simulink model "Three_Phase_Full_Wave"  (R2025b)
settings: Solver=VariableStepAuto  StartTime=0.0  StopTime=10.0  RelTol=1e-3
libraries: fl_lib x10, nesl_utility x9, ee_lib x8
settings Model: Creator=USER  LastModifiedBy=USER

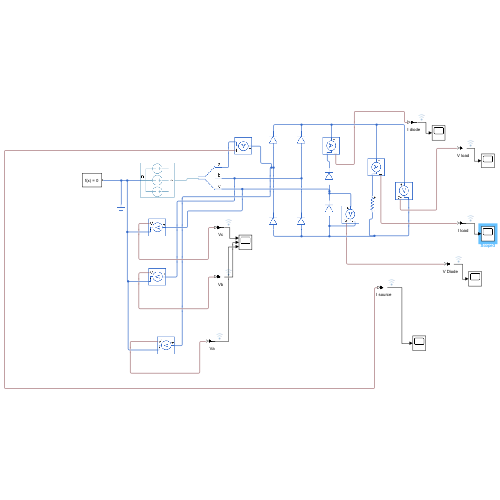
[thumbnail: Simulink's stored preview of the top-level diagram]
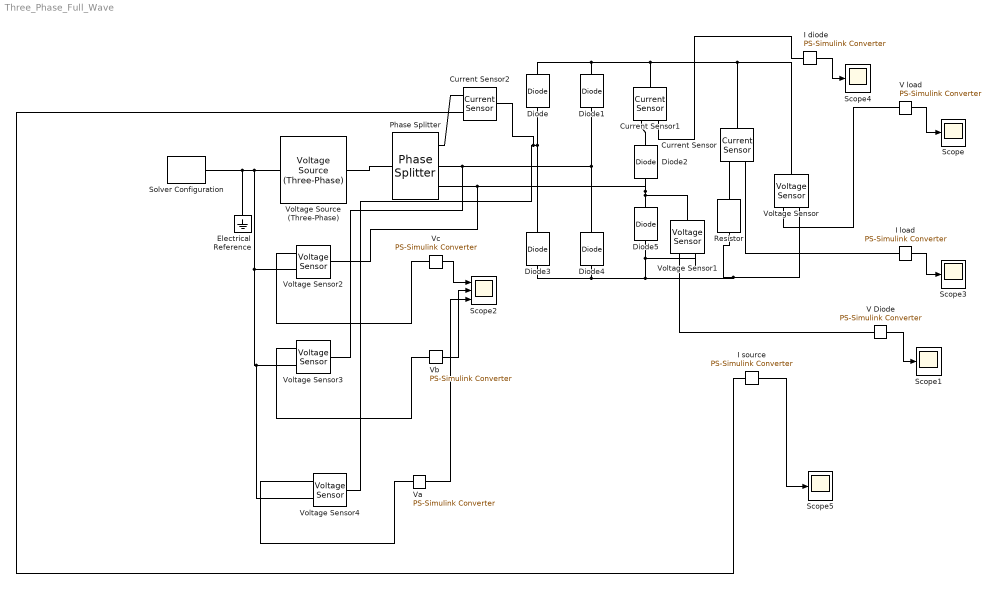
== system Three_Phase_Full_Wave ==
  Current Sensor : fl_lib/Electrical/Electrical Sensors/Current Sensor
  Current Sensor1 : fl_lib/Electrical/Electrical Sensors/Current Sensor
  Current Sensor2 : fl_lib/Electrical/Electrical Sensors/Current Sensor
  Diode{,1..5} (6 alike) : ee_lib/Semiconductors & Converters/Diode  ModelType=ee.enum.diode.modelType.pwl  TableType=ee.enum.diode.tableType.IfMat  IfMat=[.07, .12, .19, 1.75, 4.24, 7.32, 11.2; .16, .3, .72, 2.14, 5.02, 8.35, 13.12] A  VfMat=[.9, 1.15, 1.25, 1.5, 1.75, 2.17, 2.6, 2.85; .58, .68, .75, 1.1, 1.38, 1.77, 2.27, 2.7] V  TjVec=[25, 125] degC  VfVec=[.5, .7, .9, 1.3, 1.7, 2.1, 2.5] V  IfVec=[.1, .2, .5, 1, 2, 4, 7, 10] A  IrMat=[1e-06, 2e-06, 5e-06, 1e-05, 2.5e-05, 5e-05, .0001; 2e-06, 5e-06, 1e-05, 4e-05, 8e-05, .0002, .0005] A  VrMat=[10, 100, 200, 250, 300, 325, 350; 10, 70, 160, 220, 270, 300, 320] V  VrVec=[10, 20, 40, 50, 70, 80, 100] V  IrVec=[1e-06, 2e-06, 5e-06, 1e-05, 2e-05, 5e-05, .0001] A  Vf=0.6 V  Ron=0.3 Ohm  Goff=1e-8 S  prmExp=ee.enum.diode.expParam.useTwo  I12=[.0137, .545] A  V12=[.6, .7] V  RS=0 Ohm  Tmeas=298.15 K  IS=1e-12 A  ec=1  I1=0.0137 A  V1=0.6 V  N_series=1  N_parallel=1  ZenerEnable=false  Rz=0.3 Ohm  BV=inf V  C_param=ee.enum.diode.capParam.fixed  CJ=0 pF  CJ0=5 pF  Vvec=[.1, 10, 100] V  Cvec=[3.5, 1, .4] pF  VJ=1 V  Mgrad=0.5  FC=0.5  Q_param=ee.enum.diode.recoveryParam.off  iRM=-7.15 A  iF=4 A  didt=-750 A/us  trr_factor=3  trr=115 ns  Qrr=150 nA*s  Vr=-600 V  Ls=150 nH  Erec=0.03 J  TT=50 ns  tau=100 ns  T_param=ee.enum.diode.temperatureParam.off  Tdevice=298.15 K  I1_T2=0.245 A  V1_T2=0.5 V  IS_T2=1.25e-7 A  Tmeas2=125 degC  XTI_param=ee.enum.diode.xtiParam.pn  XTI=3  EG_param=ee.enum.diode.egapParam.material_si  EG=1.11 eV  dBVdT=0 V/K  enable_fault_input=simscape.enum.onoff.off  i_specify=off  i_priority=None  i=0 A  i_nominal_specify=off  i_nominal_value=1  i_nominal_unit=A  v_specify=off  v_priority=None  v=0 V  v_nominal_specify=off  v_nominal_value=1  v_nominal_unit=V  v_capacitor_specify=off  v_capacitor_priority=None  v_capacitor=0 V  v_capacitor_nominal_specify=off  v_capacitor_nominal_value=1  v_capacitor_nominal_unit=V  Qj_specify=off  Qj_priority=High  Qj=0 C  Qj_nominal_specify=off  Qj_nominal_value=1  Qj_nominal_unit=C  i_diode_specify=off  i_diode_priority=None  i_diode=0 A  i_diode_nominal_specify=off  i_diode_nominal_value=1  i_diode_nominal_unit=A  v_diode_specify=off  v_diode_priority=None  v_diode=0 V  v_diode_nominal_specify=off  v_diode_nominal_value=1  v_diode_nominal_unit=V  i_capacitor_specify=off  i_capacitor_priority=None  i_capacitor=0 A  i_capacitor_nominal_specify=off  i_capacitor_nominal_value=1  i_capacitor_nominal_unit=A  power_dissipated_specify=off  power_dissipated_priority=None  power_dissipated=0 W  power_dissipated_nominal_specify=off  power_dissipated_nominal_value=1  power_dissipated_nominal_unit=W  fidelity_level=ee.enum.diode.fidelity.includeChargeDyn  rec_loss_model=ee.enum.diode.reverseRecoveryModel.fixed  ErecVal=0 J  scaleWithIandV=true  ErecMat=zeros(2, 3) J  TjrecVec=[298.15, 398.15] K  IfrecVec=[.1, 1, 10] A  IrecVal=10 A  VrecVal=10 V  tFilter=1 / 1000 / 100 s  thermal_network_parameterization=ee.enum.thermalNetworkTopology.junctionCase  Rth=[0, 10] K/W  Rth_Cauer=[1, 3, 10] K/W  Rth_Foster=[.08, .14, .22, .16] K/W  thermal_mass_parameterization=ee.enum.thermalNetwork.timeconstant  thermal_mass=[0, 1] J/K  thermal_mass_Cauer=[.1, .3, 1] J/K  thermal_mass_Foster=[.001, .005, .05, .5] J/K  thermal_time_constant=[0, 10] s  thermal_time_constant_Cauer=[1, 3, 10] s  thermal_time_constant_Foster=[7e-05, .0007, .01, .08] s  thermal_mass_initial_temperatures=[25, 25] degC  thermal_mass_initial_temperatures_Cauer=[25, 25, 25] degC  junction_thermal_mass=0.01 J/K  Tvec_initial_Foster=[25, 25, 25, 25] degC  no_thermal_network=0  junction_temperature_specify=off  junction_temperature_priority=None  junction_temperature=25 degC  junction_temperature_nominal_specify=off  junction_temperature_nominal_value=1  junction_temperature_nominal_unit=degC
  Electrical Reference : fl_lib/Electrical/Electrical Elements/Electrical Reference
  I diode : nesl_utility/PS-Simulink Converter  PhysicalDomain=network_engine_domain  SubClassName=ps_output  LeftPortType=input  RightPortType=output  PseudoPeriodic=off  Frequencies=[]  VectorFormat=inherit  Unit=inherit  AffineConversion=off
  I load : nesl_utility/PS-Simulink Converter  PhysicalDomain=network_engine_domain  SubClassName=ps_output  LeftPortType=input  RightPortType=output  PseudoPeriodic=off  Frequencies=[]  VectorFormat=inherit  Unit=inherit  AffineConversion=off
  I source : nesl_utility/PS-Simulink Converter  PhysicalDomain=network_engine_domain  SubClassName=ps_output  LeftPortType=input  RightPortType=output  PseudoPeriodic=off  Frequencies=[]  VectorFormat=inherit  Unit=inherit  AffineConversion=off
  Phase Splitter : ee_lib/Connectors & References/Phase Splitter
  Resistor : fl_lib/Electrical/Electrical Elements/Resistor  R=200 Ohm  i_specify=off  i_priority=None  i=0 A  i_nominal_specify=off  i_nominal_value=1  i_nominal_unit=A  v_specify=off  v_priority=None  v=0 V  v_nominal_specify=off  v_nominal_value=1  v_nominal_unit=V
  Scope{,1,3..5} (5 alike) : Scope
      Scope settings: ActiveDisplayYMinimum=92.210744218018334  ActiveDisplayYMaximum=110.53269114341096
      Scope1 settings: ActiveDisplayYMinimum=-14.541376131026752  ActiveDisplayYMaximum=123.24187283383368
      Scope3 settings: ActiveDisplayYMinimum=0.45248228896029896  ActiveDisplayYMaximum=0.57237016067869884  DataLoggingVariableName=ScopeData3
      Scope4 settings: ActiveDisplayYMinimum=-14145.384322688979  ActiveDisplayYMaximum=22660.519081846294  DataLoggingVariableName=ScopeData4
      Scope5 settings: ActiveDisplayYMinimum=-14145.384322688979  ActiveDisplayYMaximum=22660.519081846294  DataLoggingVariableName=ScopeData5
  Scope2 : Scope  NumInputPorts=3
      settings: ActiveDisplayYMinimum=-79.551289054539069  ActiveDisplayYMaximum=79.551289048706238  DataLoggingVariableName=ScopeData2
  Solver Configuration : nesl_utility/Solver Configuration  PhysicalDomain=network_engine_domain  SubClassName=solver  LeftPortType=input  RightPortType=generic  Tones=[]  Harmonics=[]  SimulateNoise=off  Profile=off  UseLocalSampling=off  EnableSwitchedLinearOptims=on  FrequencyDomain=off  UseCCode=off  RelTol=0.001  AbsTol=0.001  MinStep=1e-09  ToWorkspace=off  RevertToSquareIcSolve=off  NumHomotopyIterations=100  PhasorMode=off  PhasorModeNumHarmonics=1  ConsistencySolver=NEWTON_XTOL_AFTER_FTOL  IndexReductionMethod=DerivativeReplacement  DoDC=off  ResidualTolerance=1e-09  ConsistencyTolSource=GLOBAL  ConsistencyAbsTol=0.001  ConsistencyRelTol=0.001  ConsistencyTolFactor=0.001  UseLocalSolver=off  LocalSolverChoice=NE_BACKWARD_EULER_ADVANCER  ResolveIndetEquations=on  FunctionEvalNumThread=1  LocalSolverSampleTime=0.001  DoFixedCost=off  MaxNonlinIter=3  MaxModeIter=2  ComputeImpulses=off  ImpulseIterations=2  LinearAlgebra=auto  LinearAlgebraNumThread=0  EquationFormulation=NE_TIME_EF  DelaysMemoryBudget=1024  AutomaticFiltering=on  FilteringTimeConstant=0.001  PartitionStorageMethod=AS_NEEDED  PartitionMemoryBudget=1024  PartitionMethod=ROBUST  MultibodyUseLocalSolver=off  MultibodyLocalSolverChoice=ODE1  MultibodyLocalSolverSampleTime=0.001
  V Diode : nesl_utility/PS-Simulink Converter  PhysicalDomain=network_engine_domain  SubClassName=ps_output  LeftPortType=input  RightPortType=output  PseudoPeriodic=off  Frequencies=[]  VectorFormat=inherit  Unit=inherit  AffineConversion=off
  V load : nesl_utility/PS-Simulink Converter  PhysicalDomain=network_engine_domain  SubClassName=ps_output  LeftPortType=input  RightPortType=output  PseudoPeriodic=off  Frequencies=[]  VectorFormat=inherit  Unit=inherit  AffineConversion=off
  Va : nesl_utility/PS-Simulink Converter  PhysicalDomain=network_engine_domain  SubClassName=ps_output  LeftPortType=input  RightPortType=output  PseudoPeriodic=off  Frequencies=[]  VectorFormat=inherit  Unit=inherit  AffineConversion=off
  Vb : nesl_utility/PS-Simulink Converter  PhysicalDomain=network_engine_domain  SubClassName=ps_output  LeftPortType=input  RightPortType=output  PseudoPeriodic=off  Frequencies=[]  VectorFormat=inherit  Unit=inherit  AffineConversion=off
  Vc : nesl_utility/PS-Simulink Converter  PhysicalDomain=network_engine_domain  SubClassName=ps_output  LeftPortType=input  RightPortType=output  PseudoPeriodic=off  Frequencies=[]  VectorFormat=inherit  Unit=inherit  AffineConversion=off
  Voltage Source (Three-Phase) : ee_lib/Sources/Voltage Source (Three-Phase)  vline_rms=sqrt(3)*45 V  shift=0 deg  freq=50 Hz  impedance_option=1  SShortCircuit=1e6 A*V  XR=15  R=0.01 Ohm  L=3.97e-4 H  harmonic_option=0  harmonic_orders=[5, 7, 11, 13]  harmonic_ratios=[.1, .1, .1, .1]  G_parasitic=0 1/Ohm  I_specify=off  I_priority=None  I=[0, 0, 0] A  I_nominal_specify=off  I_nominal_value=1  I_nominal_unit=A
  Voltage Sensor{,1..4} (5 alike) : fl_lib/Electrical/Electrical Sensors/Voltage Sensor
  wires:
  V load/1 -> Scope/1
  V Diode/1 -> Scope1/1
  Vc/1 -> Scope2/1
  Vb/1 -> Scope2/2
  I load/1 -> Scope3/1
  I diode/1 -> Scope4/1
  I source/1 -> Scope5/1
  Va/1 -> Scope2/3
  connections:
  Diode3/RConn1 -- Current Sensor2/LConn1 -- Voltage Sensor4/LConn1 -- Diode/LConn1
  Diode4/RConn1 -- Voltage Sensor3/LConn1 -- Phase Splitter/RConn2 -- Diode1/LConn1
  Diode5/RConn1 -- Voltage Sensor1/LConn1 -- Voltage Sensor2/LConn1 -- Phase Splitter/RConn3 -- Diode2/LConn1
  Diode5/LConn1 -- Voltage Sensor1/RConn2 -- Voltage Sensor/RConn2 -- Resistor/RConn1 -- Diode3/LConn1 -- Diode4/LConn1
  Diode1/RConn1 -- Current Sensor/LConn1 -- Voltage Sensor/LConn1 -- Current Sensor1/LConn1 -- Diode/RConn1
  Voltage Source (Three-Phase)/RConn1 -- Phase Splitter/LConn1
  Electrical Reference/LConn1 -- Voltage Sensor4/RConn2 -- Voltage Sensor3/RConn2 -- Voltage Sensor2/RConn2 -- Voltage Source (Three-Phase)/LConn1 -- Solver Configuration/RConn1
  Voltage Sensor/RConn1 -- V load/LConn1
  Voltage Sensor1/RConn1 -- V Diode/LConn1
  Voltage Sensor2/RConn1 -- Vc/LConn1
  Voltage Sensor3/RConn1 -- Vb/LConn1
  Voltage Sensor4/RConn1 -- Va/LConn1
  Current Sensor/RConn2 -- Resistor/LConn1
  Current Sensor/RConn1 -- I load/LConn1
  I diode/LConn1 -- Current Sensor1/RConn1
  Diode2/RConn1 -- Current Sensor1/RConn2
  Current Sensor2/RConn1 -- I source/LConn1
  Current Sensor2/RConn2 -- Phase Splitter/RConn1
